simulink model "SixDOFSim"  (R2026b)
settings: Solver=VariableStepAuto  StopTime=400
values from neighbouring files (symbols this model uses):
  A = [A_1 zeros(n/2,n/2);zeros(n/2,n/2) A_2]    [defineABC.m]    (also in implicit_linmod.m = -inv(E)*A_prime; nonlinear_6DOF.m = q_d*S*CA; normieren.m = Tx\A*Tx)
  B = [B_1, zeros(n/2,m/2);zeros(n/2,m/2), B_2]    [defineABC.m]    (also in implicit_linmod.m = -inv(E)*B_prime; normieren.m = Tx\B*Tu)
  C = zeros(m,n)    [defineABC.m]    (also in normieren.m = (Ty\C*Tx))
  eta_max = 10*pi/180    (= 0.174532925199)    [SixDOFModel.m]
  eta_min = - 25*pi/180    (= -0.436332312999)    [SixDOFModel.m]
  F = -inv(C*(Ak\B))    [SixDOFModel.m]    (also in coupling_controller.m = Kopt{end}; implicit_linmod.m = feval(fun, dX_ap, X_ap, U_minus))
  I_inv = inv(I)    [initializeParameters.m]
  K = lqr(sys_ol,Q,R)    [SixDOFModel.m]
  latlon_init = [0;0]    [SixDOFModel.m]
  m = size(B_1,2) + size(B_2,2)    [defineABC.m]    (also in implicit_linmod.m = length(U_ap); initializeParameters.m = 120000)
  n = size(A_1,1) +size(A_2,2)    [defineABC.m]    (also in implicit_linmod.m = length(X_ap); normieren.m = size(A,2))
  Omega_init_1 = [0;0;0]    [SixDOFModel.m]
  Omega_init_2 = [0;0;0]    [SixDOFModel.m]
  P_e_init_1 = [0;0;-h_init_1]    [SixDOFModel.m]
  P_e_init_2 = [0;0;-h_init_2]    [SixDOFModel.m]
  Phi_init_1 = [0;0;0]    [SixDOFModel.m]
  Phi_init_2 = [0;0;0]    [SixDOFModel.m]
  sigmaf_max = 10*pi/180    (= 0.174532925199)    [SixDOFModel.m]
  sigmaf_min = 0.5*pi/180    (= 0.00872664625997)    [SixDOFModel.m]
  U_ap = [U_ap_1;U_ap_2]    [SixDOFModel.m]    (also in trimValues.m = Z_ap(11:14))
  U_test = [-0.12;1;0;0;-0.1;1;0;0]    [SixDOFModel.m]
  V_init_1 = [200;0;0]    [SixDOFModel.m]
  V_init_2 = [220;0;0]    [SixDOFModel.m]
  W_ap = [X_ap_1(1); X_ap_2(1); 0; 0; X_ap_1(10); X_ap_2(10); 0; 0]    [SixDOFModel.m]
  X_ap = [X_ap_1;X_ap_2]    [SixDOFModel.m]    (also in trimValues.m = Z_ap(1:10))
  X_init = [X_init_1;X_init_2]    [SixDOFModel.m]
  xi_max = 25*pi/180    (= 0.436332312999)    [SixDOFModel.m]
  xi_min = - xi_max    (= -0.436332312999)    [SixDOFModel.m]
  zita_max = 30*pi/180    (= 0.523598775598)    [SixDOFModel.m]
  zita_min = - zita_max    (= -0.523598775598)    [SixDOFModel.m]
undefined symbols (not defined in the file or in its folder): Earth, globalParameters, nonlinear_6DOF, WGS84
libraries: aerolibfltsims x38, aerolibtransform2 x6, aerolibwind2 x2, simulink x2, aerolibatmos2 x2
(part 2 of 3)

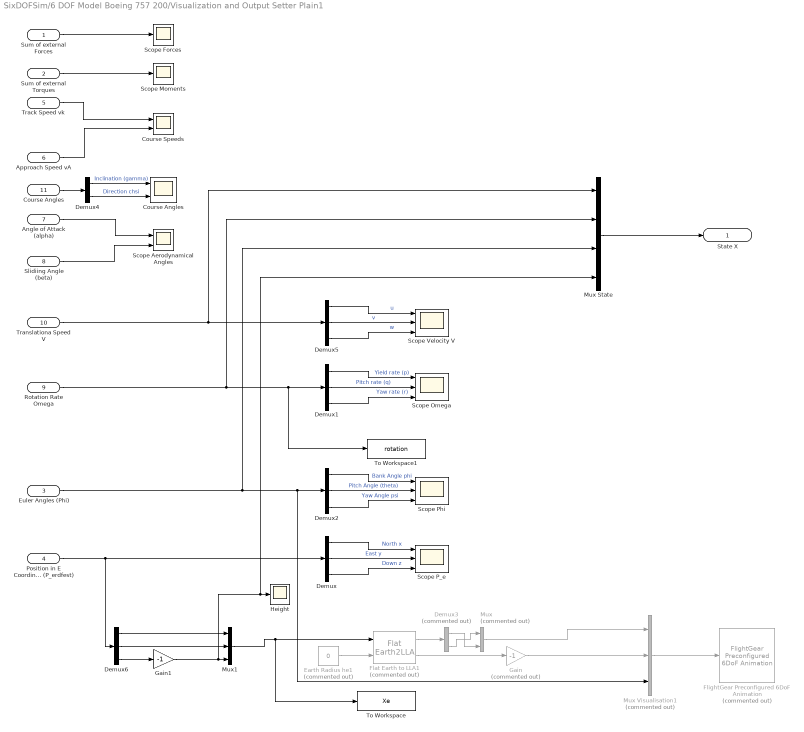
== system SixDOFSim/6 DOF Model Boeing 757 200/Visualization and Output Setter Plain1 ==
  Sum of external Forces : Inport
  Sum of external Torques : Inport  Port=2
  Euler Angles (Phi) : Inport  Port=3
  Position in E Coordinates (P_erdfest) : Inport  Port=4
  Track Speed vk : Inport  Port=5
  Approach Speed vA : Inport  Port=6
  Angle of Attack (alpha) : Inport  Port=7
  Slidiing Angle (beta) : Inport  Port=8
  Rotation Rate Omega : Inport  Port=9
  Translationa Speed V : Inport  Port=10
  "Course Angles " : Inport  Port=11
  Course Angles : Scope  NumInputPorts=2
      settings: ActiveDisplayYMinimum=-0.55672  ActiveDisplayYMaximum=0.31074  DataLoggingVariableName=ScopeData2
  Course Speeds : Scope  NumInputPorts=2
      settings: ActiveDisplayYMinimum=66.09895  ActiveDisplayYMaximum=103.76678  DataLoggingVariableName=ScopeData2
  Demux{,1..2,5..6} (5 alike) : Demux  Outputs=3
  Demux3 : Demux  Commented=on  Outputs=2
  Demux4 : Demux  Outputs=2
  Earth Radius he1 : Constant  Commented=on  Value=0
  Flat Earth to LLA1 : FlatEarth2LLA  Commented=on  R=6378137
  FlightGear Preconfigured 6DoF Animation : aerolibfltsims/FlightGear Preconfigured 6DoF Animation  Commented=on  xFlightGearVersion=v2019.1  DestinationIpAddress=127.0.0.1  DestinationPort=5502  SampleTime=1/30  packetVersion=24
  Gain : Gain  Commented=on  Gain=-1
  Gain1 : Gain  Gain=-1
  Height : Scope
      settings: ActiveDisplayYMinimum=7438.34389  ActiveDisplayYMaximum=8064.45716  DataLoggingVariableName=ScopeData4
  Mux : Mux  Commented=on  Inputs=2
  Mux State : Mux
  Mux Visualisation1 : Mux  Commented=on  Inputs=3
  Mux1 : Mux  Inputs=3
  Scope Aerodynamical Angles : Scope  NumInputPorts=2
      settings: ActiveDisplayYMinimum=-0.32941  ActiveDisplayYMaximum=0.05301  DataLoggingVariableName=ScopeData6
  Scope Forces : Scope
      settings: ActiveDisplayYMinimum=-9.65264854834E+6  ActiveDisplayYMaximum=3.78260201913E+6
  Scope Moments : Scope
      settings: ActiveDisplayYMinimum=-635313.46804  ActiveDisplayYMaximum=300416.0741  DataLoggingVariableName=ScopeData2
  Scope Omega : Scope  NumInputPorts=3
      settings: ActiveDisplayYMinimum=-0.09538  ActiveDisplayYMaximum=0.05227  DataLoggingVariableName=ScopeData3
  Scope P_e : Scope  NumInputPorts=3
      settings: ActiveDisplayYMinimum=-406.67749  ActiveDisplayYMaximum=3660.09739  DataLoggingVariableName=ScopeData5
  Scope Phi : Scope  NumInputPorts=3
      settings: ActiveDisplayYMinimum=-0.4812  ActiveDisplayYMaximum=0.12125  DataLoggingVariableName=ScopeData4
  Scope Velocity V : Scope  NumInputPorts=3
      settings: ActiveDisplayYMinimum=-86.24132  ActiveDisplayYMaximum=231.80459  DataLoggingVariableName=ScopeData3
  To Workspace : ToWorkspace  VariableName=Xe  SaveFormat=Timeseries  SampleTime=-1
  To Workspace1 : ToWorkspace  VariableName=rotation  SaveFormat=Timeseries  SampleTime=-1
  State X : Outport
  wires:
  Mux State/1 -> State X/1
  Demux1/2 -> Scope Omega/2  "Pitch rate (q)"
  Demux2/2 -> Scope Phi/2  "Pitch Angle (theta)"
  Demux1/3 -> Scope Omega/3  "Yaw rate (r)"
  Demux1/1 -> Scope Omega/1  "Yield rate (p)"
  Demux2/1 -> Scope Phi/1  "Bank Angle phi"
  Demux/1 -> Scope P_e/1  "North x"
  Demux/2 -> Scope P_e/2  "East y"
  Demux/3 -> Scope P_e/3  "Down z"
  Demux2/3 -> Scope Phi/3  "Yaw Angle psi"
  Demux3/1 -> Mux/2
  Demux3/2 -> Mux/1
  Mux Visualisation1/1 -> FlightGear Preconfigured 6DoF Animation/1
  Flat Earth to LLA1/1 -> Demux3/1
  Earth Radius he1/1 -> Flat Earth to LLA1/2
  Mux/1 -> Mux Visualisation1/1
  Track Speed vk/1 -> Course Speeds/1
  Approach Speed vA/1 -> Course Speeds/2
  Sum of external Forces/1 -> Scope Forces/1
  Sum of external Torques/1 -> Scope Moments/1
  Demux4/1 -> Course Angles/1  "Inclination (gamma)"
  Demux4/2 -> Course Angles/2  "Direction chsi"
  "Course Angles "/1 -> Demux4/1
  Angle of Attack (alpha)/1 -> Scope Aerodynamical Angles/1
  Slidiing Angle (beta)/1 -> Scope Aerodynamical Angles/2
  Position in E Coordinates (P_erdfest)/1 -> Demux6/1, Demux/1
  Flat Earth to LLA1/2 -> Gain/1
  Gain/1 -> Mux Visualisation1/2
  Euler Angles (Phi)/1 -> Mux Visualisation1/3, Demux2/1, Mux State/3
  Rotation Rate Omega/1 -> To Workspace1/1, Demux1/1, Mux State/2
  Demux5/3 -> Scope Velocity V/3  "w"
  Demux5/1 -> Scope Velocity V/1  "u"
  Demux5/2 -> Scope Velocity V/2  "v"
  Translationa Speed V/1 -> Demux5/1, Mux State/1
  Demux6/3 -> Gain1/1
  Gain1/1 -> Mux State/4, Height/1, Mux1/3
  Demux6/1 -> Mux1/1
  Demux6/2 -> Mux1/2
  Mux1/1 -> To Workspace/1, Flat Earth to LLA1/1

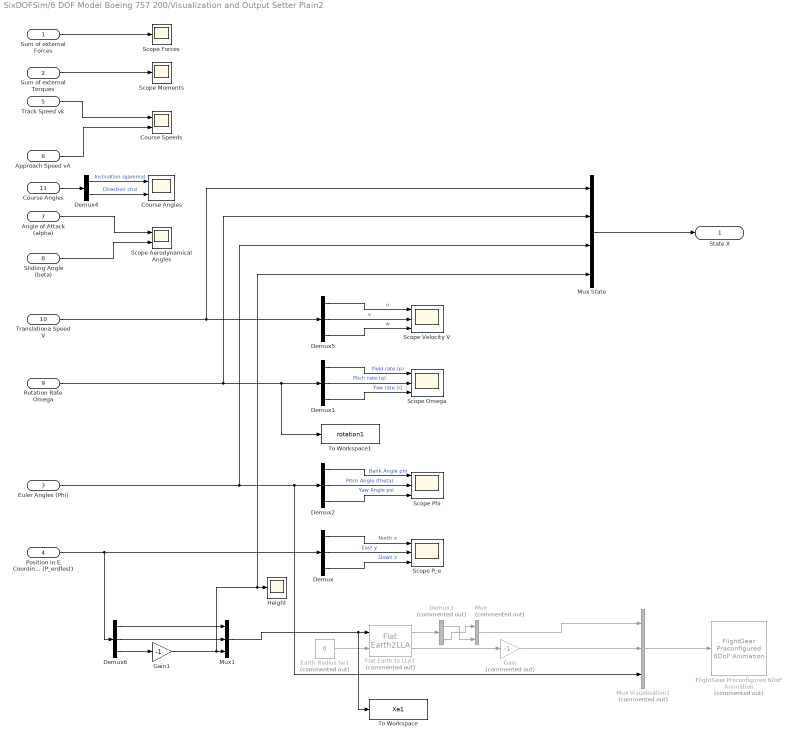
== system SixDOFSim/6 DOF Model Boeing 757 200/Visualization and Output Setter Plain2 ==
  Sum of external Forces : Inport
  Sum of external Torques : Inport  Port=2
  Euler Angles (Phi) : Inport  Port=3
  Position in E Coordinates (P_erdfest) : Inport  Port=4
  Track Speed vk : Inport  Port=5
  Approach Speed vA : Inport  Port=6
  Angle of Attack (alpha) : Inport  Port=7
  Slidiing Angle (beta) : Inport  Port=8
  Rotation Rate Omega : Inport  Port=9
  Translationa Speed V : Inport  Port=10
  "Course Angles " : Inport  Port=11
  Course Angles : Scope  NumInputPorts=2
      settings: ActiveDisplayYMinimum=-0.6798  ActiveDisplayYMaximum=0.51288  DataLoggingVariableName=ScopeData2
  Course Speeds : Scope  NumInputPorts=2
      settings: ActiveDisplayYMinimum=66.09895  ActiveDisplayYMaximum=103.76678  DataLoggingVariableName=ScopeData2
  Demux{,1..2,5..6} (5 alike) : Demux  Outputs=3
  Demux3 : Demux  Commented=on  Outputs=2
  Demux4 : Demux  Outputs=2
  Earth Radius he1 : Constant  Commented=on  Value=0
  Flat Earth to LLA1 : FlatEarth2LLA  Commented=on  R=6378137
  FlightGear Preconfigured 6DoF Animation : aerolibfltsims/FlightGear Preconfigured 6DoF Animation  Commented=on  xFlightGearVersion=v2019.1  DestinationIpAddress=127.0.0.1  DestinationPort=5502  SampleTime=1/30  packetVersion=24
  Gain : Gain  Commented=on  Gain=-1
  Gain1 : Gain  Gain=-1
  Height : Scope
      settings: ActiveDisplayYMinimum=7558.66984  ActiveDisplayYMaximum=8063.70802  DataLoggingVariableName=ScopeData4
  Mux : Mux  Commented=on  Inputs=2
  Mux State : Mux
  Mux Visualisation1 : Mux  Commented=on  Inputs=3
  Mux1 : Mux  Inputs=3
  Scope Aerodynamical Angles : Scope  NumInputPorts=2
      settings: ActiveDisplayYMinimum=-0.32941  ActiveDisplayYMaximum=0.05301  DataLoggingVariableName=ScopeData6
  Scope Forces : Scope
      settings: ActiveDisplayYMinimum=-9.65264854834E+6  ActiveDisplayYMaximum=3.78260201913E+6
  Scope Moments : Scope
      settings: ActiveDisplayYMinimum=-651410.77127  ActiveDisplayYMaximum=638305.54031  DataLoggingVariableName=ScopeData2
  Scope Omega : Scope  NumInputPorts=3
      settings: ActiveDisplayYMinimum=-0.50231  ActiveDisplayYMaximum=0.11601  DataLoggingVariableName=ScopeData3
  Scope P_e : Scope  NumInputPorts=3
      settings: ActiveDisplayYMinimum=-182.69972  ActiveDisplayYMaximum=1644.29749  DataLoggingVariableName=ScopeData5
  Scope Phi : Scope  NumInputPorts=3
      settings: ActiveDisplayYMinimum=-0.67619  ActiveDisplayYMaximum=0.30731  DataLoggingVariableName=ScopeData4
  Scope Velocity V : Scope  NumInputPorts=3
      settings: ActiveDisplayYMinimum=-26.68463  ActiveDisplayYMaximum=140.16169  DataLoggingVariableName=ScopeData3
  To Workspace : ToWorkspace  VariableName=Xe1  SaveFormat=Timeseries  SampleTime=-1
  To Workspace1 : ToWorkspace  VariableName=rotation1  SaveFormat=Timeseries  SampleTime=-1
  State X : Outport
  wires:
  Mux State/1 -> State X/1
  Demux1/2 -> Scope Omega/2  "Pitch rate (q)"
  Demux2/2 -> Scope Phi/2  "Pitch Angle (theta)"
  Demux1/3 -> Scope Omega/3  "Yaw rate (r)"
  Demux1/1 -> Scope Omega/1  "Yield rate (p)"
  Demux2/1 -> Scope Phi/1  "Bank Angle phi"
  Demux/1 -> Scope P_e/1  "North x"
  Demux/2 -> Scope P_e/2  "East y"
  Demux/3 -> Scope P_e/3  "Down z"
  Demux2/3 -> Scope Phi/3  "Yaw Angle psi"
  Demux3/1 -> Mux/2
  Demux3/2 -> Mux/1
  Mux Visualisation1/1 -> FlightGear Preconfigured 6DoF Animation/1
  Flat Earth to LLA1/1 -> Demux3/1
  Earth Radius he1/1 -> Flat Earth to LLA1/2
  Mux/1 -> Mux Visualisation1/1
  Track Speed vk/1 -> Course Speeds/1
  Approach Speed vA/1 -> Course Speeds/2
  Sum of external Forces/1 -> Scope Forces/1
  Sum of external Torques/1 -> Scope Moments/1
  Demux4/1 -> Course Angles/1  "Inclination (gamma)"
  Demux4/2 -> Course Angles/2  "Direction chsi"
  "Course Angles "/1 -> Demux4/1
  Angle of Attack (alpha)/1 -> Scope Aerodynamical Angles/1
  Slidiing Angle (beta)/1 -> Scope Aerodynamical Angles/2
  Position in E Coordinates (P_erdfest)/1 -> Demux6/1, Demux/1
  Flat Earth to LLA1/2 -> Gain/1
  Gain/1 -> Mux Visualisation1/2
  Euler Angles (Phi)/1 -> Mux Visualisation1/3, Demux2/1, Mux State/3
  Rotation Rate Omega/1 -> To Workspace1/1, Demux1/1, Mux State/2
  Demux5/3 -> Scope Velocity V/3  "w"
  Demux5/1 -> Scope Velocity V/1  "u"
  Demux5/2 -> Scope Velocity V/2  "v"
  Translationa Speed V/1 -> Demux5/1, Mux State/1
  Demux6/3 -> Gain1/1
  Gain1/1 -> Mux State/4, Height/1, Mux1/3
  Demux6/1 -> Mux1/1
  Demux6/2 -> Mux1/2
  Mux1/1 -> To Workspace/1, Flat Earth to LLA1/1

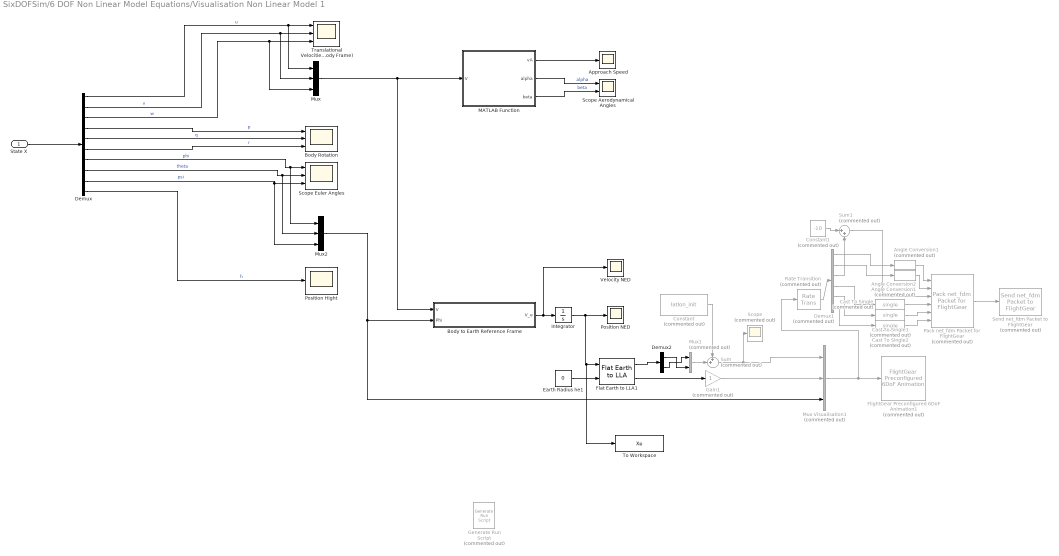
== system SixDOFSim/6 DOF Non Linear Model Equations/Visualisation Non Linear Model 1 ==
  State X : Inport
  Angle Conversion1 : aerolibfltsims/FlightGear Preconfigured 6DoF Animation/Angle Conversion1  Commented=on  SystemSampleTime=-1  VariantActivationTime=update diagram  Latency=0  AutoFrameSizeCalculation=off
  Angle Conversion2 : aerolibfltsims/FlightGear Preconfigured 6DoF Animation/Angle Conversion1  Commented=on  SystemSampleTime=-1  VariantActivationTime=update diagram  Latency=0  AutoFrameSizeCalculation=off
  Approach Speed : Scope
      settings: ActiveDisplayYMinimum=90.717446245698  ActiveDisplayYMaximum=90.71744624575  DataLoggingVariableName=ScopeData5
  Body Rotation : Scope  NumInputPorts=3
      settings: ActiveDisplayYMinimum=-4.9E-13  ActiveDisplayYMaximum=1.7E-13  DataLoggingVariableName=ScopeData4
  "Body to Earth Reference Frame " : MATLAB Function  TreatAsAtomicUnit=on
  Cast To Single : DataTypeConversion  Commented=on  OutDataTypeStr=single  SaturateOnIntegerOverflow=off  RndMeth=Floor
  Cast To Single1 : DataTypeConversion  Commented=on  OutDataTypeStr=single  SaturateOnIntegerOverflow=off  RndMeth=Floor
  Cast To Single2 : DataTypeConversion  Commented=on  OutDataTypeStr=single  SaturateOnIntegerOverflow=off  RndMeth=Floor
  Constant : Constant  Commented=on  Value=latlon_init
  Constant1 : Constant  Commented=on  Value=-10
  Demux : Demux  Outputs=10
  Demux1 : Demux  Commented=on  Outputs=6
  Demux2 : Demux  Outputs=2
  Earth Radius he1 : Constant  Value=0
  Flat Earth to LLA1 : aerolibtransform2/Flat Earth to LLA  units=Metric (MKS)  ptype=Earth (WGS84)  F=1/298.257223563  R=6378137  refPosPort=off  LL0=[0 10]  psi=0
  FlightGear Preconfigured 6DoF Animation1 : aerolibfltsims/FlightGear Preconfigured 6DoF Animation  Commented=on  xFlightGearVersion=v2019.1  DestinationIpAddress=127.0.0.1  DestinationPort=5502  SampleTime=1/30  packetVersion=24
  Gain1 : Gain  Commented=on
  Generate Run Script : aerolibfltsims/Generate Run Script  Commented=on  Architecture=Win64  dataFlow=Send  GeometryModelName=c172p  AirportId=KSFO  RunwayId=10L  InitialAltitude=7224  InitialHeading=113  OffsetDistance=4.72  OffsetAzimuth=0  InstallScenery=off  DisableShaders=on  OriginAddress=127.0.0.1  DestinationPort=5502  OriginPort=5505  LocalAddress=127.0.0.1  OutputFileName=runfg.bat  FlightGearBaseDirectory=D:\Flight Gear\FlightGear 2018.1.1
  Integrator : Integrator  InitialCondition=P_e_init_1
  MATLAB Function : MATLAB Function  TreatAsAtomicUnit=on
  Mux : Mux  Inputs=3
  Mux Visualisation1 : Mux  Commented=on  Inputs=3
  Mux1 : Mux  Commented=on  Inputs=2
  Mux2 : Mux  Inputs=3
  Pack net_fdm Packet for FlightGear : aerolibfltsims/Pack net_fdm Packet for FlightGear  Commented=on  FlightGearVersion=v2019.1  ShowPositionAttitudeInputs=on  ShowVelocityAccelerationInputs=off  ShowControlSurfacePositionInputs=off  ShowEngineFuelInputs=off  ShowLandingGearInputs=off  ShowEnvironmentInputs=off  SampleTime=1/30  packetVersion=24
  Position Hight : Scope
      settings: ActiveDisplayYMinimum=7481.53398  ActiveDisplayYMaximum=8060.37764  DataLoggingVariableName=ScopeData2
  Position NED : Scope
      settings: ActiveDisplayYMinimum=-15.3099  ActiveDisplayYMaximum=3.98752
  Rate Transition : RateTransition  Commented=on  Integrity=off  Deterministic=off
  Scope : Scope  Commented=on
      settings: ActiveDisplayYMinimum=9.99999999993  ActiveDisplayYMaximum=10.00000000031  DataLoggingVariableName=ScopeData7
  Scope Aerodynamical Angles : Scope  NumInputPorts=2
      settings: ActiveDisplayYMinimum=-0.00068  ActiveDisplayYMaximum=0.00608
  Scope Euler Angles : Scope  NumInputPorts=3
      settings: ActiveDisplayYMinimum=-0.50414  ActiveDisplayYMaximum=0.14503  DataLoggingVariableName=ScopeData3
  Send net_fdm Packet to FlightGear : aerolibfltsims/Send net_fdm Packet to FlightGear  Commented=on  DestinationIpAddress=127.0.0.1  DestinationPort=5503  LocalIpPort=-1  varLen=off  SampleTime=1/30
  Sum : Sum  Commented=on  Inputs=++|
  Sum1 : Sum  Commented=on  Inputs=|++
  To Workspace : ToWorkspace  VariableName=Xe  SaveFormat=Timeseries  SampleTime=-1
  Translational Velocities (Body Frame) : Scope  NumInputPorts=3
      settings: ActiveDisplayYMinimum=-98.50656  ActiveDisplayYMaximum=233.1674
  Velocity NED : Scope
      settings: ActiveDisplayYMinimum=-11.33968  ActiveDisplayYMaximum=102.05713  DataLoggingVariableName=ScopeData2
  wires:
  State X/1 -> Demux/1
  Demux2/2 -> Mux1/1
  Flat Earth to LLA1/2 -> Gain1/1
  Gain1/1 -> Mux Visualisation1/2
  Mux Visualisation1/1 -> FlightGear Preconfigured 6DoF Animation1/1, Rate Transition/1
  Earth Radius he1/1 -> Flat Earth to LLA1/2
  Flat Earth to LLA1/1 -> Demux2/1
  Demux2/1 -> Mux1/2
  "Body to Earth Reference Frame "/1(V_e) -> Velocity NED/1, Integrator/1
  Integrator/1 -> Position NED/1, To Workspace/1, Flat Earth to LLA1/1
  Demux/1 -> Mux/1, Translational Velocities (Body Frame)/1  "u"
  Demux/2 -> Mux/2, Translational Velocities (Body Frame)/2  "v"
  Demux/3 -> Translational Velocities (Body Frame)/3, Mux/3  "w"
  Demux/4 -> Body Rotation/1  "p"
  Demux/5 -> Body Rotation/2  "q"
  Demux/6 -> Body Rotation/3  "r"
  Demux/7 -> Mux2/1, Scope Euler Angles/1  "phi"
  Demux/8 -> Mux2/2, Scope Euler Angles/2  "theta"
  Demux/9 -> Mux2/3, Scope Euler Angles/3  "psi"
  Demux/10 -> Position Hight/1  "h"
  Mux/1 -> MATLAB Function/1(V), "Body to Earth Reference Frame "/1(V)
  Mux2/1 -> "Body to Earth Reference Frame "/2(Phi), Mux Visualisation1/3
  MATLAB Function/1(vA) -> Approach Speed/1
  MATLAB Function/2(alpha) -> Scope Aerodynamical Angles/1  "alpha"
  MATLAB Function/3(beta) -> Scope Aerodynamical Angles/2  "beta"
  Mux1/1 -> Sum/2
  Sum/1 -> Scope/1, Mux Visualisation1/1
  Constant/1 -> Sum/1
  Pack net_fdm Packet for FlightGear/1 -> Send net_fdm Packet to FlightGear/1
  Angle Conversion1/1 -> Pack net_fdm Packet for FlightGear/1
  Angle Conversion2/1 -> Pack net_fdm Packet for FlightGear/2
  Cast To Single/1 -> Pack net_fdm Packet for FlightGear/4
  Cast To Single1/1 -> Pack net_fdm Packet for FlightGear/5
  Cast To Single2/1 -> Pack net_fdm Packet for FlightGear/6
  Demux1/2 -> Angle Conversion2/1
  Rate Transition/1 -> Demux1/1
  Demux1/1 -> Angle Conversion1/1
  Constant1/1 -> Sum1/1
  Demux1/3 -> Sum1/2
  Sum1/1 -> Pack net_fdm Packet for FlightGear/3
  Demux1/4 -> Cast To Single/1
  Demux1/5 -> Cast To Single1/1
  Demux1/6 -> Cast To Single2/1

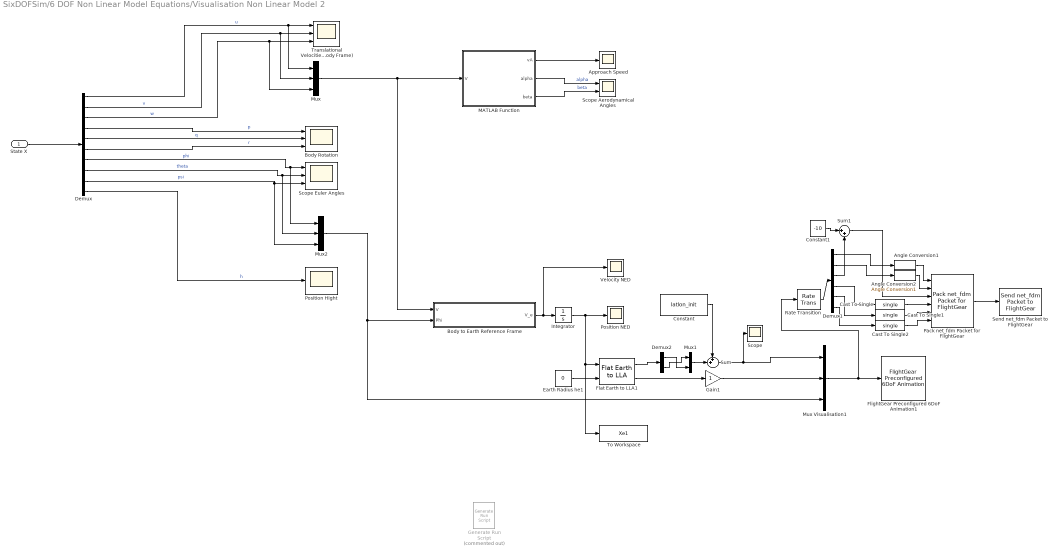
== system SixDOFSim/6 DOF Non Linear Model Equations/Visualisation Non Linear Model 2 ==
  State X : Inport
  Angle Conversion1 : aerolibfltsims/FlightGear Preconfigured 6DoF Animation/Angle Conversion1  SystemSampleTime=-1  VariantActivationTime=update diagram  Latency=0  AutoFrameSizeCalculation=off
  Angle Conversion2 : aerolibfltsims/FlightGear Preconfigured 6DoF Animation/Angle Conversion1  SystemSampleTime=-1  VariantActivationTime=update diagram  Latency=0  AutoFrameSizeCalculation=off
  Approach Speed : Scope
      settings: ActiveDisplayYMinimum=90.717446245698  ActiveDisplayYMaximum=90.71744624575  DataLoggingVariableName=ScopeData5
  Body Rotation : Scope  NumInputPorts=3
      settings: ActiveDisplayYMinimum=-4.9E-13  ActiveDisplayYMaximum=1.7E-13  DataLoggingVariableName=ScopeData4
  "Body to Earth Reference Frame " : MATLAB Function  TreatAsAtomicUnit=on
  Cast To Single : DataTypeConversion  OutDataTypeStr=single  SaturateOnIntegerOverflow=off  RndMeth=Floor
  Cast To Single1 : DataTypeConversion  OutDataTypeStr=single  SaturateOnIntegerOverflow=off  RndMeth=Floor
  Cast To Single2 : DataTypeConversion  OutDataTypeStr=single  SaturateOnIntegerOverflow=off  RndMeth=Floor
  Constant : Constant  Value=latlon_init
  Constant1 : Constant  Value=-10
  Demux : Demux  Outputs=10
  Demux1 : Demux  Outputs=6
  Demux2 : Demux  Outputs=2
  Earth Radius he1 : Constant  Value=0
  Flat Earth to LLA1 : aerolibtransform2/Flat Earth to LLA  units=Metric (MKS)  ptype=Earth (WGS84)  F=1/298.257223563  R=6378137  refPosPort=off  LL0=[0 10]  psi=0
  FlightGear Preconfigured 6DoF Animation1 : aerolibfltsims/FlightGear Preconfigured 6DoF Animation  xFlightGearVersion=v2019.1  DestinationIpAddress=127.0.0.1  DestinationPort=5502  SampleTime=1/30  packetVersion=24
  Gain1 : Gain
  Generate Run Script : aerolibfltsims/Generate Run Script  Commented=on  Architecture=Win64  dataFlow=Send  GeometryModelName=c172p  AirportId=KSFO  RunwayId=10L  InitialAltitude=7224  InitialHeading=113  OffsetDistance=4.72  OffsetAzimuth=0  InstallScenery=off  DisableShaders=on  OriginAddress=127.0.0.1  DestinationPort=5502  OriginPort=5505  LocalAddress=127.0.0.1  OutputFileName=runfg.bat  FlightGearBaseDirectory=D:\Flight Gear\FlightGear 2018.1.1
  Integrator : Integrator  InitialCondition=P_e_init_2
  MATLAB Function : MATLAB Function  TreatAsAtomicUnit=on
  Mux : Mux  Inputs=3
  Mux Visualisation1 : Mux  Inputs=3
  Mux1 : Mux  Inputs=2
  Mux2 : Mux  Inputs=3
  Pack net_fdm Packet for FlightGear : aerolibfltsims/Pack net_fdm Packet for FlightGear  FlightGearVersion=v2019.1  ShowPositionAttitudeInputs=on  ShowVelocityAccelerationInputs=off  ShowControlSurfacePositionInputs=off  ShowEngineFuelInputs=off  ShowLandingGearInputs=off  ShowEnvironmentInputs=off  SampleTime=1/30  packetVersion=24
  Position Hight : Scope
      settings: ActiveDisplayYMinimum=-141.15664  ActiveDisplayYMaximum=1137.90629  DataLoggingVariableName=ScopeData2
  Position NED : Scope
      settings: ActiveDisplayYMinimum=-1351.79362  ActiveDisplayYMaximum=2166.14254
  Rate Transition : RateTransition  Integrity=off  Deterministic=off
  Scope : Scope
      settings: ActiveDisplayYMinimum=9.99999999993  ActiveDisplayYMaximum=10.00000000031  DataLoggingVariableName=ScopeData7
  Scope Aerodynamical Angles : Scope  NumInputPorts=2
      settings: ActiveDisplayYMinimum=-0.00068  ActiveDisplayYMaximum=0.00608
  Scope Euler Angles : Scope  NumInputPorts=3
      settings: ActiveDisplayYMinimum=-0.69993  ActiveDisplayYMaximum=0.52973  DataLoggingVariableName=ScopeData3
  Send net_fdm Packet to FlightGear : aerolibfltsims/Send net_fdm Packet to FlightGear  DestinationIpAddress=127.0.0.1  DestinationPort=5503  LocalIpPort=-1  varLen=off  SampleTime=1/30
  Sum : Sum  Inputs=++|
  Sum1 : Sum  Inputs=|++
  To Workspace : ToWorkspace  VariableName=Xe1  SaveFormat=Timeseries  SampleTime=-1
  Translational Velocities (Body Frame) : Scope  NumInputPorts=3
      settings: ActiveDisplayYMinimum=-30.67675  ActiveDisplayYMaximum=164.16583
  Velocity NED : Scope
      settings: ActiveDisplayYMinimum=-11.33968  ActiveDisplayYMaximum=102.05713  DataLoggingVariableName=ScopeData2
  wires:
  State X/1 -> Demux/1
  Demux2/2 -> Mux1/1
  Flat Earth to LLA1/2 -> Gain1/1
  Gain1/1 -> Mux Visualisation1/2
  Mux Visualisation1/1 -> FlightGear Preconfigured 6DoF Animation1/1, Rate Transition/1
  Earth Radius he1/1 -> Flat Earth to LLA1/2
  Flat Earth to LLA1/1 -> Demux2/1
  Demux2/1 -> Mux1/2
  "Body to Earth Reference Frame "/1(V_e) -> Velocity NED/1, Integrator/1
  Integrator/1 -> Position NED/1, To Workspace/1, Flat Earth to LLA1/1
  Demux/1 -> Mux/1, Translational Velocities (Body Frame)/1  "u"
  Demux/2 -> Mux/2, Translational Velocities (Body Frame)/2  "v"
  Demux/3 -> Translational Velocities (Body Frame)/3, Mux/3  "w"
  Demux/4 -> Body Rotation/1  "p"
  Demux/5 -> Body Rotation/2  "q"
  Demux/6 -> Body Rotation/3  "r"
  Demux/7 -> Mux2/1, Scope Euler Angles/1  "phi"
  Demux/8 -> Mux2/2, Scope Euler Angles/2  "theta"
  Demux/9 -> Mux2/3, Scope Euler Angles/3  "psi"
  Demux/10 -> Position Hight/1  "h"
  Mux/1 -> MATLAB Function/1(V), "Body to Earth Reference Frame "/1(V)
  Mux2/1 -> "Body to Earth Reference Frame "/2(Phi), Mux Visualisation1/3
  MATLAB Function/1(vA) -> Approach Speed/1
  MATLAB Function/2(alpha) -> Scope Aerodynamical Angles/1  "alpha"
  MATLAB Function/3(beta) -> Scope Aerodynamical Angles/2  "beta"
  Mux1/1 -> Sum/2
  Sum/1 -> Scope/1, Mux Visualisation1/1
  Constant/1 -> Sum/1
  Pack net_fdm Packet for FlightGear/1 -> Send net_fdm Packet to FlightGear/1
  Angle Conversion1/1 -> Pack net_fdm Packet for FlightGear/1
  Angle Conversion2/1 -> Pack net_fdm Packet for FlightGear/2
  Cast To Single/1 -> Pack net_fdm Packet for FlightGear/4
  Cast To Single1/1 -> Pack net_fdm Packet for FlightGear/5
  Cast To Single2/1 -> Pack net_fdm Packet for FlightGear/6
  Demux1/2 -> Angle Conversion2/1
  Rate Transition/1 -> Demux1/1
  Demux1/1 -> Angle Conversion1/1
  Constant1/1 -> Sum1/1
  Demux1/3 -> Sum1/2
  Sum1/1 -> Pack net_fdm Packet for FlightGear/3
  Demux1/4 -> Cast To Single/1
  Demux1/5 -> Cast To Single1/1
  Demux1/6 -> Cast To Single2/1

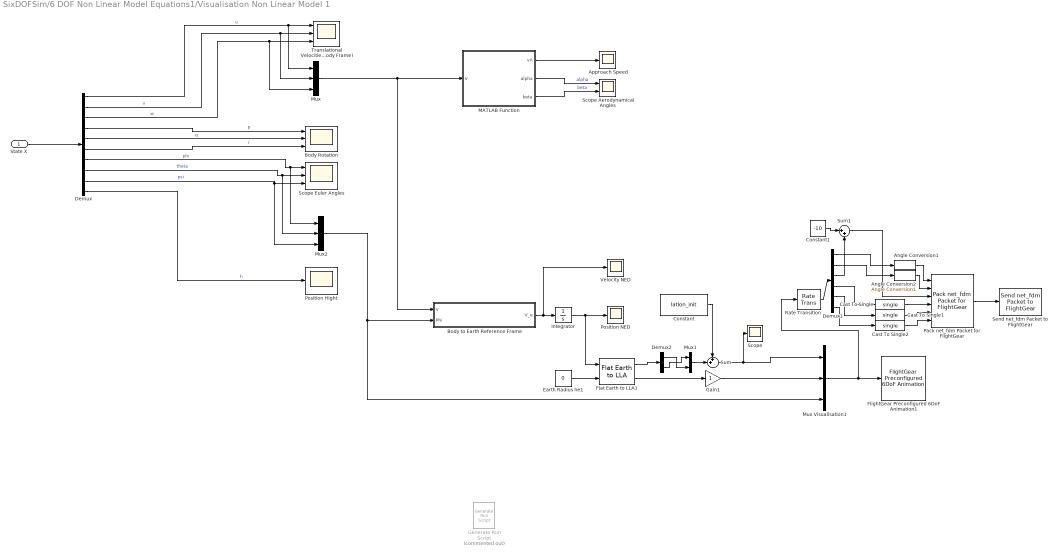
== system SixDOFSim/6 DOF Non Linear Model Equations1/Visualisation Non Linear Model 1 ==
  State X : Inport
  Angle Conversion1 : aerolibfltsims/FlightGear Preconfigured 6DoF Animation/Angle Conversion1  SystemSampleTime=-1  VariantActivationTime=update diagram  Latency=0  AutoFrameSizeCalculation=off
  Angle Conversion2 : aerolibfltsims/FlightGear Preconfigured 6DoF Animation/Angle Conversion1  SystemSampleTime=-1  VariantActivationTime=update diagram  Latency=0  AutoFrameSizeCalculation=off
  Approach Speed : Scope
      settings: ActiveDisplayYMinimum=90.717446245698  ActiveDisplayYMaximum=90.71744624575  DataLoggingVariableName=ScopeData5
  Body Rotation : Scope  NumInputPorts=3
      settings: ActiveDisplayYMinimum=-4.9E-13  ActiveDisplayYMaximum=1.7E-13  DataLoggingVariableName=ScopeData4
  "Body to Earth Reference Frame " : MATLAB Function  TreatAsAtomicUnit=on
  Cast To Single : DataTypeConversion  OutDataTypeStr=single  SaturateOnIntegerOverflow=off  RndMeth=Floor
  Cast To Single1 : DataTypeConversion  OutDataTypeStr=single  SaturateOnIntegerOverflow=off  RndMeth=Floor
  Cast To Single2 : DataTypeConversion  OutDataTypeStr=single  SaturateOnIntegerOverflow=off  RndMeth=Floor
  Constant : Constant  Value=latlon_init
  Constant1 : Constant  Value=-10
  Demux : Demux  Outputs=10
  Demux1 : Demux  Outputs=6
  Demux2 : Demux  Outputs=2
  Earth Radius he1 : Constant  Value=0
  Flat Earth to LLA1 : aerolibtransform2/Flat Earth to LLA  units=Metric (MKS)  ptype=Earth (WGS84)  F=1/298.257223563  R=6378137  refPosPort=off  LL0=[0 10]  psi=0
  FlightGear Preconfigured 6DoF Animation1 : aerolibfltsims/FlightGear Preconfigured 6DoF Animation  xFlightGearVersion=v2019.1  DestinationIpAddress=127.0.0.1  DestinationPort=5502  SampleTime=1/30  packetVersion=24
  Gain1 : Gain
  Generate Run Script : aerolibfltsims/Generate Run Script  Commented=on  Architecture=Win64  dataFlow=Send  GeometryModelName=c172p  AirportId=KSFO  RunwayId=10L  InitialAltitude=7224  InitialHeading=113  OffsetDistance=4.72  OffsetAzimuth=0  InstallScenery=off  DisableShaders=on  OriginAddress=127.0.0.1  DestinationPort=5502  OriginPort=5505  LocalAddress=127.0.0.1  OutputFileName=runfg.bat  FlightGearBaseDirectory=D:\Flight Gear\FlightGear 2018.1.1
  Integrator : Integrator  InitialCondition=P_e_init_1
  MATLAB Function : MATLAB Function  TreatAsAtomicUnit=on
  Mux : Mux  Inputs=3
  Mux Visualisation1 : Mux  Inputs=3
  Mux1 : Mux  Inputs=2
  Mux2 : Mux  Inputs=3
  Pack net_fdm Packet for FlightGear : aerolibfltsims/Pack net_fdm Packet for FlightGear  FlightGearVersion=v2019.1  ShowPositionAttitudeInputs=on  ShowVelocityAccelerationInputs=off  ShowControlSurfacePositionInputs=off  ShowEngineFuelInputs=off  ShowLandingGearInputs=off  ShowEnvironmentInputs=off  SampleTime=1/30  packetVersion=24
  Position Hight : Scope
      settings: ActiveDisplayYMinimum=233.96265  ActiveDisplayYMaximum=1085.11526  DataLoggingVariableName=ScopeData2
  Position NED : Scope
      settings: ActiveDisplayYMinimum=-1569.88178  ActiveDisplayYMaximum=4128.93604
  Rate Transition : RateTransition  Integrity=off  Deterministic=off
  Scope : Scope
      settings: ActiveDisplayYMinimum=9.99999999993  ActiveDisplayYMaximum=10.00000000031  DataLoggingVariableName=ScopeData7
  Scope Aerodynamical Angles : Scope  NumInputPorts=2
      settings: ActiveDisplayYMinimum=-0.00068  ActiveDisplayYMaximum=0.00608
  Scope Euler Angles : Scope  NumInputPorts=3
      settings: ActiveDisplayYMinimum=-0.67463  ActiveDisplayYMaximum=0.49342  DataLoggingVariableName=ScopeData3
  Send net_fdm Packet to FlightGear : aerolibfltsims/Send net_fdm Packet to FlightGear  DestinationIpAddress=127.0.0.1  DestinationPort=5503  LocalIpPort=-1  varLen=off  SampleTime=1/30
  Sum : Sum  Inputs=++|
  Sum1 : Sum  Inputs=|++
  Translational Velocities (Body Frame) : Scope  NumInputPorts=3
      settings: ActiveDisplayYMinimum=-5.714  ActiveDisplayYMaximum=7.05401
  Velocity NED : Scope
      settings: ActiveDisplayYMinimum=-11.33968  ActiveDisplayYMaximum=102.05713  DataLoggingVariableName=ScopeData2
  wires:
  State X/1 -> Demux/1
  Demux2/2 -> Mux1/1
  Flat Earth to LLA1/2 -> Gain1/1
  Gain1/1 -> Mux Visualisation1/2
  Mux Visualisation1/1 -> FlightGear Preconfigured 6DoF Animation1/1, Rate Transition/1
  Earth Radius he1/1 -> Flat Earth to LLA1/2
  Flat Earth to LLA1/1 -> Demux2/1
  Demux2/1 -> Mux1/2
  "Body to Earth Reference Frame "/1(V_e) -> Velocity NED/1, Integrator/1
  Integrator/1 -> Position NED/1, Flat Earth to LLA1/1
  Demux/1 -> Mux/1, Translational Velocities (Body Frame)/1  "u"
  Demux/2 -> Mux/2, Translational Velocities (Body Frame)/2  "v"
  Demux/3 -> Translational Velocities (Body Frame)/3, Mux/3  "w"
  Demux/4 -> Body Rotation/1  "p"
  Demux/5 -> Body Rotation/2  "q"
  Demux/6 -> Body Rotation/3  "r"
  Demux/7 -> Mux2/1, Scope Euler Angles/1  "phi"
  Demux/8 -> Mux2/2, Scope Euler Angles/2  "theta"
  Demux/9 -> Mux2/3, Scope Euler Angles/3  "psi"
  Demux/10 -> Position Hight/1  "h"
  Mux/1 -> MATLAB Function/1(V), "Body to Earth Reference Frame "/1(V)
  Mux2/1 -> "Body to Earth Reference Frame "/2(Phi), Mux Visualisation1/3
  MATLAB Function/1(vA) -> Approach Speed/1
  MATLAB Function/2(alpha) -> Scope Aerodynamical Angles/1  "alpha"
  MATLAB Function/3(beta) -> Scope Aerodynamical Angles/2  "beta"
  Mux1/1 -> Sum/2
  Sum/1 -> Scope/1, Mux Visualisation1/1
  Constant/1 -> Sum/1
  Pack net_fdm Packet for FlightGear/1 -> Send net_fdm Packet to FlightGear/1
  Angle Conversion1/1 -> Pack net_fdm Packet for FlightGear/1
  Angle Conversion2/1 -> Pack net_fdm Packet for FlightGear/2
  Cast To Single/1 -> Pack net_fdm Packet for FlightGear/4
  Cast To Single1/1 -> Pack net_fdm Packet for FlightGear/5
  Cast To Single2/1 -> Pack net_fdm Packet for FlightGear/6
  Demux1/2 -> Angle Conversion2/1
  Rate Transition/1 -> Demux1/1
  Demux1/1 -> Angle Conversion1/1
  Constant1/1 -> Sum1/1
  Demux1/3 -> Sum1/2
  Sum1/1 -> Pack net_fdm Packet for FlightGear/3
  Demux1/4 -> Cast To Single/1
  Demux1/5 -> Cast To Single1/1
  Demux1/6 -> Cast To Single2/1

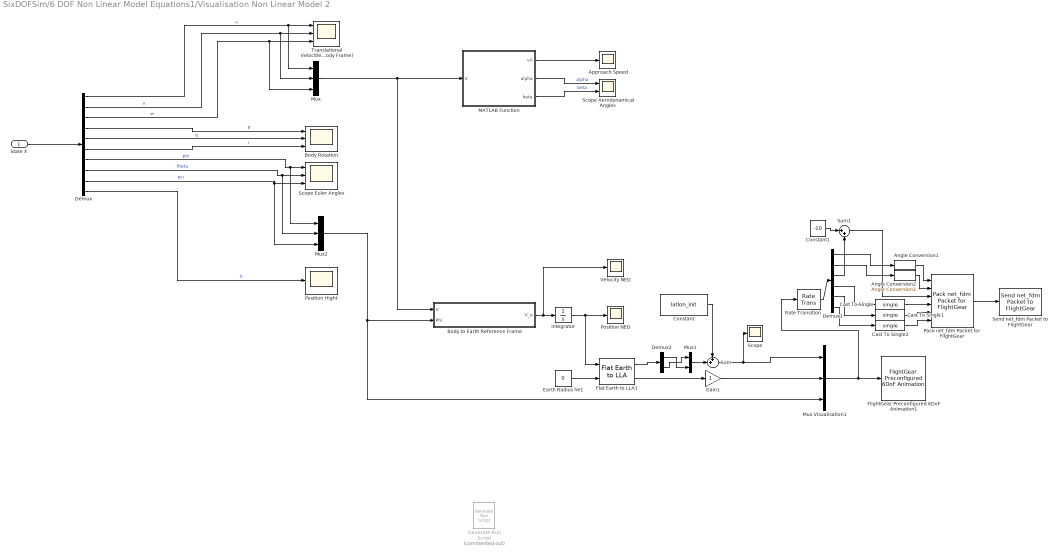
== system SixDOFSim/6 DOF Non Linear Model Equations1/Visualisation Non Linear Model 2 ==
  State X : Inport
  Angle Conversion1 : aerolibfltsims/FlightGear Preconfigured 6DoF Animation/Angle Conversion1  SystemSampleTime=-1  VariantActivationTime=update diagram  Latency=0  AutoFrameSizeCalculation=off
  Angle Conversion2 : aerolibfltsims/FlightGear Preconfigured 6DoF Animation/Angle Conversion1  SystemSampleTime=-1  VariantActivationTime=update diagram  Latency=0  AutoFrameSizeCalculation=off
  Approach Speed : Scope
      settings: ActiveDisplayYMinimum=90.717446245698  ActiveDisplayYMaximum=90.71744624575  DataLoggingVariableName=ScopeData5
  Body Rotation : Scope  NumInputPorts=3
      settings: ActiveDisplayYMinimum=-4.9E-13  ActiveDisplayYMaximum=1.7E-13  DataLoggingVariableName=ScopeData4
  "Body to Earth Reference Frame " : MATLAB Function  TreatAsAtomicUnit=on
  Cast To Single : DataTypeConversion  OutDataTypeStr=single  SaturateOnIntegerOverflow=off  RndMeth=Floor
  Cast To Single1 : DataTypeConversion  OutDataTypeStr=single  SaturateOnIntegerOverflow=off  RndMeth=Floor
  Cast To Single2 : DataTypeConversion  OutDataTypeStr=single  SaturateOnIntegerOverflow=off  RndMeth=Floor
  Constant : Constant  Value=latlon_init
  Constant1 : Constant  Value=-10
  Demux : Demux  Outputs=10
  Demux1 : Demux  Outputs=6
  Demux2 : Demux  Outputs=2
  Earth Radius he1 : Constant  Value=0
  Flat Earth to LLA1 : aerolibtransform2/Flat Earth to LLA  units=Metric (MKS)  ptype=Earth (WGS84)  F=1/298.257223563  R=6378137  refPosPort=off  LL0=[0 10]  psi=0
  FlightGear Preconfigured 6DoF Animation1 : aerolibfltsims/FlightGear Preconfigured 6DoF Animation  xFlightGearVersion=v2019.1  DestinationIpAddress=127.0.0.1  DestinationPort=5502  SampleTime=1/30  packetVersion=24
  Gain1 : Gain
  Generate Run Script : aerolibfltsims/Generate Run Script  Commented=on  Architecture=Win64  dataFlow=Send  GeometryModelName=c172p  AirportId=KSFO  RunwayId=10L  InitialAltitude=7224  InitialHeading=113  OffsetDistance=4.72  OffsetAzimuth=0  InstallScenery=off  DisableShaders=on  OriginAddress=127.0.0.1  DestinationPort=5502  OriginPort=5505  LocalAddress=127.0.0.1  OutputFileName=runfg.bat  FlightGearBaseDirectory=D:\Flight Gear\FlightGear 2018.1.1
  Integrator : Integrator  InitialCondition=P_e_init_2
  MATLAB Function : MATLAB Function  TreatAsAtomicUnit=on
  Mux : Mux  Inputs=3
  Mux Visualisation1 : Mux  Inputs=3
  Mux1 : Mux  Inputs=2
  Mux2 : Mux  Inputs=3
  Pack net_fdm Packet for FlightGear : aerolibfltsims/Pack net_fdm Packet for FlightGear  FlightGearVersion=v2019.1  ShowPositionAttitudeInputs=on  ShowVelocityAccelerationInputs=off  ShowControlSurfacePositionInputs=off  ShowEngineFuelInputs=off  ShowLandingGearInputs=off  ShowEnvironmentInputs=off  SampleTime=1/30  packetVersion=24
  Position Hight : Scope
      settings: ActiveDisplayYMinimum=-141.15664  ActiveDisplayYMaximum=1137.90629  DataLoggingVariableName=ScopeData2
  Position NED : Scope
      settings: ActiveDisplayYMinimum=-1351.79362  ActiveDisplayYMaximum=2166.14254
  Rate Transition : RateTransition  Integrity=off  Deterministic=off
  Scope : Scope
      settings: ActiveDisplayYMinimum=9.99999999993  ActiveDisplayYMaximum=10.00000000031  DataLoggingVariableName=ScopeData7
  Scope Aerodynamical Angles : Scope  NumInputPorts=2
      settings: ActiveDisplayYMinimum=-0.00068  ActiveDisplayYMaximum=0.00608
  Scope Euler Angles : Scope  NumInputPorts=3
      settings: ActiveDisplayYMinimum=-0.69993  ActiveDisplayYMaximum=0.52973  DataLoggingVariableName=ScopeData3
  Send net_fdm Packet to FlightGear : aerolibfltsims/Send net_fdm Packet to FlightGear  DestinationIpAddress=127.0.0.1  DestinationPort=5503  LocalIpPort=-1  varLen=off  SampleTime=1/30
  Sum : Sum  Inputs=++|
  Sum1 : Sum  Inputs=|++
  Translational Velocities (Body Frame) : Scope  NumInputPorts=3
      settings: ActiveDisplayYMinimum=-30.67675  ActiveDisplayYMaximum=164.16583
  Velocity NED : Scope
      settings: ActiveDisplayYMinimum=-11.33968  ActiveDisplayYMaximum=102.05713  DataLoggingVariableName=ScopeData2
  wires:
  State X/1 -> Demux/1
  Demux2/2 -> Mux1/1
  Flat Earth to LLA1/2 -> Gain1/1
  Gain1/1 -> Mux Visualisation1/2
  Mux Visualisation1/1 -> FlightGear Preconfigured 6DoF Animation1/1, Rate Transition/1
  Earth Radius he1/1 -> Flat Earth to LLA1/2
  Flat Earth to LLA1/1 -> Demux2/1
  Demux2/1 -> Mux1/2
  "Body to Earth Reference Frame "/1(V_e) -> Velocity NED/1, Integrator/1
  Integrator/1 -> Position NED/1, Flat Earth to LLA1/1
  Demux/1 -> Mux/1, Translational Velocities (Body Frame)/1  "u"
  Demux/2 -> Mux/2, Translational Velocities (Body Frame)/2  "v"
  Demux/3 -> Translational Velocities (Body Frame)/3, Mux/3  "w"
  Demux/4 -> Body Rotation/1  "p"
  Demux/5 -> Body Rotation/2  "q"
  Demux/6 -> Body Rotation/3  "r"
  Demux/7 -> Mux2/1, Scope Euler Angles/1  "phi"
  Demux/8 -> Mux2/2, Scope Euler Angles/2  "theta"
  Demux/9 -> Mux2/3, Scope Euler Angles/3  "psi"
  Demux/10 -> Position Hight/1  "h"
  Mux/1 -> MATLAB Function/1(V), "Body to Earth Reference Frame "/1(V)
  Mux2/1 -> "Body to Earth Reference Frame "/2(Phi), Mux Visualisation1/3
  MATLAB Function/1(vA) -> Approach Speed/1
  MATLAB Function/2(alpha) -> Scope Aerodynamical Angles/1  "alpha"
  MATLAB Function/3(beta) -> Scope Aerodynamical Angles/2  "beta"
  Mux1/1 -> Sum/2
  Sum/1 -> Scope/1, Mux Visualisation1/1
  Constant/1 -> Sum/1
  Pack net_fdm Packet for FlightGear/1 -> Send net_fdm Packet to FlightGear/1
  Angle Conversion1/1 -> Pack net_fdm Packet for FlightGear/1
  Angle Conversion2/1 -> Pack net_fdm Packet for FlightGear/2
  Cast To Single/1 -> Pack net_fdm Packet for FlightGear/4
  Cast To Single1/1 -> Pack net_fdm Packet for FlightGear/5
  Cast To Single2/1 -> Pack net_fdm Packet for FlightGear/6
  Demux1/2 -> Angle Conversion2/1
  Rate Transition/1 -> Demux1/1
  Demux1/1 -> Angle Conversion1/1
  Constant1/1 -> Sum1/1
  Demux1/3 -> Sum1/2
  Sum1/1 -> Pack net_fdm Packet for FlightGear/3
  Demux1/4 -> Cast To Single/1
  Demux1/5 -> Cast To Single1/1
  Demux1/6 -> Cast To Single2/1

== system SixDOFSim/6 DOF Model Boeing 757 200/Motion model Plain1/Dynamics ==
  Forces : Inport
  Torque : Inport  Port=2
  Euler Angles( Phi) : Inport  Port=3
  Divide : Product  Inputs=*/
  Dynamics Forces Feedback : MATLAB Function  TreatAsAtomicUnit=on
  Dynamics Torque Feedback : MATLAB Function  TreatAsAtomicUnit=on
  Gain : Gain  Gain=I_inv  Multiplication=Matrix(K*u) (u vector)
  Integrator Omega 1 : Integrator  InitialCondition=Omega_init_1
  Integrator V 1 : Integrator  InitialCondition=V_init_1
  Sum : Sum  Inputs=-+|+
  Sum1 : Sum  Inputs=|+-
  Total mass of plaiin 1 (Betanker) : Subsystem
  Transformation of gravity in (Körperfestes System) : MATLAB Function  TreatAsAtomicUnit=on
  Rotation Rate Omega : Outport
  Translational Speed V : Outport  Port=2
  wires:
  Euler Angles( Phi)/1 -> Transformation of gravity in (Körperfestes System)/1(Phi)
  Transformation of gravity in (Körperfestes System)/1(gravityAcceleration) -> Sum/3
  Forces/1 -> Divide/1
  Sum/1 -> Integrator V 1/1
  Integrator V 1/1 -> Translational Speed V/1, Dynamics Forces Feedback/2(V)
  Divide/1 -> Sum/2
  Dynamics Forces Feedback/1(acceleration) -> Sum/1
  Torque/1 -> Sum1/1
  Sum1/1 -> Gain/1
  Gain/1 -> Integrator Omega 1/1
  Integrator Omega 1/1 -> Dynamics Forces Feedback/1(Omega), Dynamics Torque Feedback/1(Omega), Rotation Rate Omega/1
  Dynamics Torque Feedback/1(torqueFeedback) -> Sum1/2
  Total mass of plaiin 1 (Betanker)/1(m_total) -> Divide/2

== system SixDOFSim/6 DOF Model Boeing 757 200/Motion model Plain1/Kinematics ==
  Omega : Inport
  V : Inport  Port=2
  Gain : Gain  Gain=eye(3)  Multiplication=Matrix(K*u) (u vector)
  Gain1 : Gain  Gain=eye(3)  Multiplication=Matrix(K*u) (u vector)
  Integrator P_erdfest : Integrator  InitialCondition=P_e_init_1
  Integrator Phi : Integrator  InitialCondition=Phi_init_1
  Rotation Rate of the g-System : MATLAB Function  TreatAsAtomicUnit=on
  Velocity Transformation to Erdfestkoordinaten : MATLAB Function  TreatAsAtomicUnit=on
  Euler Angle (Phi) : Outport
  P_erdfest : Outport  Port=2
  wires:
  Integrator P_erdfest/1 -> P_erdfest/1  "P_DEN"
  Velocity Transformation to Erdfestkoordinaten/1(velocityDEN) -> Gain/1  "V_DEN"
  V/1 -> Velocity Transformation to Erdfestkoordinaten/2(V)
  Rotation Rate of the g-System/1(dPhi) -> Integrator Phi/1
  Gain/1 -> Integrator P_erdfest/1
  Omega/1 -> Rotation Rate of the g-System/1(Omega)
  Integrator Phi/1 -> Gain1/1
  Gain1/1 -> Rotation Rate of the g-System/2(Phi), Velocity Transformation to Erdfestkoordinaten/1(Phi), Euler Angle (Phi)/1

== system SixDOFSim/6 DOF Model Boeing 757 200/Motion model Plain2 /Dynamics ==
  Torque : Inport
  Forces : Inport  Port=2
  Euler Angles( Phi) : Inport  Port=3
  Divide : Product  Inputs=*/
  Dynamics Forces Feedback : MATLAB Function  TreatAsAtomicUnit=on
  Dynamics Torque Feedback : MATLAB Function  TreatAsAtomicUnit=on
  Gain : Gain  Gain=I_inv  Multiplication=Matrix(K*u) (u vector)
  Integrator Omega : Integrator  InitialCondition=Omega_init_2
  Integrator V : Integrator  InitialCondition=V_init_2
  Scope : Scope
      settings: ActiveDisplayYMinimum=20000  ActiveDisplayYMaximum=220000
  Sum : Sum  Inputs=-+|+
  Sum1 : Sum  Inputs=|+-
  Total mass of plain 2 (being refueled) : Subsystem
  Transformation of gravity in (Körperfestes System) : MATLAB Function  TreatAsAtomicUnit=on
  Rotation Rate Omega : Outport
  Translational Speed V : Outport  Port=2
  wires:
  Euler Angles( Phi)/1 -> Transformation of gravity in (Körperfestes System)/1(Phi)
  Transformation of gravity in (Körperfestes System)/1(gravityAcceleration) -> Sum/3
  Sum/1 -> Integrator V/1
  Integrator V/1 -> Translational Speed V/1, Dynamics Forces Feedback/2(V)
  Dynamics Forces Feedback/1(acceleration) -> Sum/1
  Torque/1 -> Sum1/1
  Sum1/1 -> Gain/1
  Gain/1 -> Integrator Omega/1
  Integrator Omega/1 -> Dynamics Forces Feedback/1(Omega), Dynamics Torque Feedback/1(Omega), Rotation Rate Omega/1
  Dynamics Torque Feedback/1(torqueFeedback) -> Sum1/2
  Forces/1 -> Divide/1
  Divide/1 -> Sum/2
  Total mass of plain 2 (being refueled)/1(Total Mass) -> Scope/1, Divide/2

== system SixDOFSim/6 DOF Model Boeing 757 200/Motion model Plain2 /Kinematics ==
  Omega : Inport
  V : Inport  Port=2
  Gain : Gain  Gain=eye(3)  Multiplication=Matrix(K*u) (u vector)
  Gain1 : Gain  Gain=eye(3)  Multiplication=Matrix(K*u) (u vector)
  Integrator P_erdfest : Integrator  InitialCondition=P_e_init_2
  Integrator Phi : Integrator  InitialCondition=Phi_init_2
  Rotation Rate of the g-System : MATLAB Function  TreatAsAtomicUnit=on
  Velocity Transformation to Erdfestkoordinaten : MATLAB Function  TreatAsAtomicUnit=on
  Euler Angle (Phi) : Outport
  P_erdfest : Outport  Port=2
  wires:
  Integrator P_erdfest/1 -> P_erdfest/1  "P_DEN"
  Velocity Transformation to Erdfestkoordinaten/1(velocityDEN) -> Gain/1  "V_DEN"
  V/1 -> Velocity Transformation to Erdfestkoordinaten/2(V)
  Rotation Rate of the g-System/1(dPhi) -> Integrator Phi/1
  Gain/1 -> Integrator P_erdfest/1
  Omega/1 -> Rotation Rate of the g-System/1(Omega)
  Integrator Phi/1 -> Gain1/1
  Gain1/1 -> Rotation Rate of the g-System/2(Phi), Velocity Transformation to Erdfestkoordinaten/1(Phi), Euler Angle (Phi)/1

== system SixDOFSim/6 DOF Model Boeing 757 200/Motion model Plain1/Dynamics/Total mass of plaiin 1 (Betanker) ==
  Constant : Constant  Value=m+globalParameters.m_fuel
  Constant1 : Constant  Value=0
  Constant2 : Constant  Value=globalParameters.refuel
  Ramp : simulink/Sources/Ramp  slope=globalParameters.m_fuel/globalParameters.time_refuel  start=globalParameters.start_time_refuel  InitialOutput=0  VectorParams1D=off
  Saturation : Saturate  UpperLimit=globalParameters.m_fuel  LowerLimit=0
  Sum2 : Sum  Inputs=|+-
  Switch : Switch  Criteria=u2 > Threshold  SaturateOnIntegerOverflow=off  InputSameDT=off
  m_total : Outport
  wires:
  Switch/1 -> Sum2/2
  Constant2/1 -> Switch/2
  Ramp/1 -> Saturation/1
  Saturation/1 -> Switch/3
  Constant1/1 -> Switch/1
  Constant/1 -> Sum2/1
  Sum2/1 -> m_total/1

== system SixDOFSim/6 DOF Model Boeing 757 200/Motion model Plain2 /Dynamics/Total mass of plain 2 (being refueled) ==
  Constant : Constant  Value=m
  Constant1 : Constant  Value=0
  Constant2 : Constant  Value=globalParameters.refuel
  Ramp : simulink/Sources/Ramp  slope=globalParameters.m_fuel/globalParameters.time_refuel  start=globalParameters.start_time_refuel  InitialOutput=0
  Saturation : Saturate  UpperLimit=globalParameters.m_fuel  LowerLimit=0
  Sum2 : Sum  Inputs=|++
  Switch : Switch  Criteria=u2 > Threshold  SaturateOnIntegerOverflow=off  InputSameDT=off
  Total Mass : Outport
  wires:
  Switch/1 -> Sum2/2
  Sum2/1 -> Total Mass/1
  Saturation/1 -> Switch/3
  Constant/1 -> Sum2/1
  Ramp/1 -> Saturation/1
  Constant2/1 -> Switch/2
  Constant1/1 -> Switch/1

== matlab function SixDOFSim/6 DOF Linear/Visualisation Non Linear Model Plain 2/Body to Earth Reference Frame  ==
  data: V input; Phi input; V_e output
function V_e = getEarthPosition(V,Phi)

Tfg = coordTransfMatrix(Phi(1),1)*coordTransfMatrix(Phi(2),2)*coordTransfMatrix(Phi(3),3); % Transformation Matrix goedetic --> body reference Frame
Tgf = Tfg';
V_e = Tgf*V;
V_e(3) =  V_e(3);

== matlab function SixDOFSim/6 DOF Linear/Visualisation Non Linear Model Plain 2/MATLAB Function ==
  data: V input; vA output; alpha output; beta output
function [vA,alpha,beta] = getAerodynamical(V)
u = V(1);
v = V(2);
w = V(3);
vA = sqrt(u^2+v^2+w^2);
alpha = atan2(w,u);
beta = asin(v/vA);

== matlab function SixDOFSim/6 DOF Model Boeing 757 200/Forces and Moments Plane 1/Thrust Force and Torque ==
  data: sigmaf input; Rf output; globalParameters parameter; Qf output
function [Rf,Qf] = thrust(sigmaf,globalParameters)
%Get Thrus Force Rf and Thrust Moment Qf
%sigmaf: Throttle Position [rad]
P_thrust =globalParameters.P_thrust;
i_f =globalParameters.i_f;
F_max = globalParameters.Fmax;

F_res = F_max*sigmaf; %Resultant Force Absolute Value
Rf = F_res*[cos(i_f);0;sin(i_f)]; %Thrust Force 
P_thrust_tilde = vecToMat(P_thrust);
Qf = P_thrust_tilde*Rf; %Thrust Moment

== matlab function SixDOFSim/6 DOF Model Boeing 757 200/Geometrical Coefficients Plane 1/Geometrie Rotational Coefficients ==
  data: vA input; alpha input; beta input; Omega input; eta input; zita input; globalParameters parameter; xi input; CL output; CM output; CN output
function [CL,CM,CN] = torqueGeometricCoefficient(vA,alpha,beta,Omega,eta,zita, globalParameters,xi)
%eta = Höheruderwinkel (elevator) [rad]
%zita = Seitenruderwinkel (ruder) [rad]
%xi = Querruderwinkel (Airlon) [rad]
%Global Parameters
lt = globalParameters.lt;
S = globalParameters.S;
St = globalParameters.St;
c = globalParameters.c;
alpha_L0 = -11.5*pi/180;
gradient_alpha_epsolon = 0.25;
epsolon = gradient_alpha_epsolon*(alpha - alpha_L0); %Downwash [rad]
%Moments Coefficients
N = [-1.4*beta;-0.59-3.1*(St*lt/(c*S))*(alpha-epsolon);(1-alpha*(180/(15*pi)))*beta]; %Static Moments Effects
Jakobi_CM_X = (c/vA)*[-11,    0,           5;
                      0,-4.03*St*lt^2/(S*c^2),0;
                      1.7,          0   , -11.5];
Jakobi_CM_U = [-0.6, 0, 0.22;
               0,    -3.1*St*lt/(S*c),0;
               0, 0, -0.63];      % Dependence of Control Variables
           
C_torque = N + Jakobi_CM_X*Omega + Jakobi_CM_U*[xi;eta;zita];
CL = C_torque(1);
CM = C_torque(2);
CN = C_torque(3);

== matlab function SixDOFSim/6 DOF Model Boeing 757 200/Forces and Moments Plain2/Aerodynamical Forces ==
  data: CA input; RA output; CW input; CQ input; vA input; alpha input; beta input; rho input; globalParameters parameter
function RA = getAerodynForces(CA,CW,CQ,vA, alpha, beta, rho,globalParameters)
%[~,~,~,rho] = atmosisa(h); %Air density 
q_d = 0.5*vA^2*rho; %Dynamic Preassure
S = globalParameters.S ;


A = q_d*S*CA; %Lift Force [N]
W = q_d*S*CW; %Air Resistance [N]
Q = q_d*S*CQ; %Transverse Force [N]

Tfa = coordTransfMatrix(alpha,2)*coordTransfMatrix(-beta,3); %Transformation Matrix Aerodynamics -> Körperfest

RA_a =[-W;Q;-A];
RA = Tfa*RA_a;

== matlab function SixDOFSim/6 DOF Model Boeing 757 200/Forces and Moments Plain2/Aerodynamical Torque ==
  data: RA input; CL input; QA output size=3; CM input; CN input; vA input; globalParameters parameter; rho input
function QA = getAerodynTorque(RA,CL,CM,CN, vA, globalParameters,rho)
%Aircraft Parameters
b = globalParameters.b;
c = globalParameters.c;
S = globalParameters.S;
P_centerGravity = globalParameters.P_centerGravity;
P_aerodynCenter = globalParameters.P_aerodynCenter;
q_d = 0.5*vA^2*rho; %Dynamic Preassure
QA = zeros(3,1);
QA_aerodynCenter = q_d*S*[0.5*b*CL;c*CM;0.5*b*CN];
QA = QA_aerodynCenter + vecToMat(P_centerGravity- P_aerodynCenter)*RA;

== matlab function SixDOFSim/6 DOF Model Boeing 757 200/Forces and Moments Plain2/Thrust Force and Torque ==
  data: sigmaf input; Rf output; globalParameters parameter; Qf output
function [Rf,Qf] = thrust(sigmaf,globalParameters)
%Get Thrus Force Rf and Thrust Moment Qf
%sigmaf: Throttle Position [rad]
P_thrust =globalParameters.P_thrust;
i_f =globalParameters.i_f;
F_max = globalParameters.Fmax;

F_res = F_max*sigmaf; %Resultant Force Absolute Value
Rf = F_res*[cos(i_f);0;sin(i_f)]; %Thrust Force 
P_thrust_tilde = vecToMat(P_thrust);
Qf = P_thrust_tilde*Rf; %Thrust Moment

== matlab function SixDOFSim/6 DOF Model Boeing 757 200/Motion model Plain2 /Dynamics/Dynamics Forces Feedback ==
  data: Omega input; V input; acceleration output; globalParameters parameter
function acceleration = accelerationFeedback(Omega,V,globalParameters)
Omega_e_tilde = globalParameters.Omega_e_tilde;
Omega_tilde = vecToMat(Omega);
acceleration = (Omega_tilde + Omega_e_tilde)*V;

== matlab function SixDOFSim/6 DOF Model Boeing 757 200/Motion model Plain2 /Dynamics/Dynamics Torque Feedback ==
  data: Omega input; torqueFeedback output; globalParameters parameter
function torqueFeedback = getTorqueFeedback(Omega,globalParameters)
I = globalParameters.I;
Omega_tilde = vecToMat(Omega);
help = Omega_tilde*I;
torqueFeedback = help*Omega;

== matlab function SixDOFSim/6 DOF Model Boeing 757 200/Geometrical Coefficients Plain2/Geometrie Rotational Coefficients ==
  data: vA input; alpha input; beta input; Omega input; eta input; zita input; globalParameters parameter; xi input; CL output; CM output; CN output
function [CL,CM,CN] = torqueGeometricCoefficient(vA,alpha,beta,Omega,eta,zita, globalParameters,xi)
%eta = Höheruderwinkel (elevator) [rad]
%zita = Seitenruderwinkel (ruder) [rad]
%xi = Querruderwinkel (Airlon) [rad]
%Global Parameters
lt = globalParameters.lt;
S = globalParameters.S;
St = globalParameters.St;
c = globalParameters.c;
alpha_L0 = -11.5*pi/180;
gradient_alpha_epsolon = 0.25;
epsolon = gradient_alpha_epsolon*(alpha - alpha_L0); %Downwash [rad]
%Moments Coefficients
N = [-1.4*beta;-0.59-3.1*(St*lt/(c*S))*(alpha-epsolon);(1-alpha*(180/(15*pi)))*beta]; %Static Moments Effects
Jakobi_CM_X = (c/vA)*[-11,    0,           5;
                      0,-4.03*St*lt^2/(S*c^2),0;
                      1.7,          0   , -11.5];
Jakobi_CM_U = [-0.6, 0, 0.22;
               0,    -3.1*St*lt/(S*c),0;
               0, 0, -0.63];      % Dependence of Control Variables
           
C_torque = N + Jakobi_CM_X*Omega + Jakobi_CM_U*[xi;eta;zita];
CL = C_torque(1);
CM = C_torque(2);
CN = C_torque(3);
